simulink model "Local_In"  (R2025b)
settings: Solver=VariableStepAuto  StartTime=0.0  StopTime=10.0  RelTol=1e-3
settings Model: Creator=EMK7KOR  LastModifiedBy=CAQ2KOR

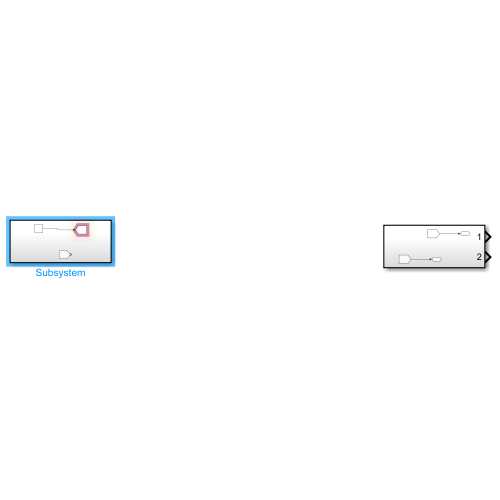
[thumbnail: Simulink's stored preview of the top-level diagram]
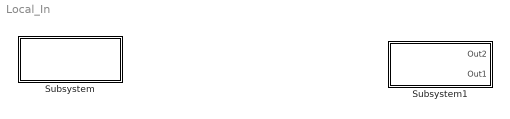
== system Local_In ==
  Subsystem : Subsystem
  Subsystem1 : Subsystem

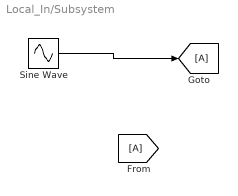
== system Local_In/Subsystem ==
  From : From
  Goto : Goto
  Sine Wave : Sin  SampleTime=0
  wires:
  Sine Wave/1 -> Goto/1

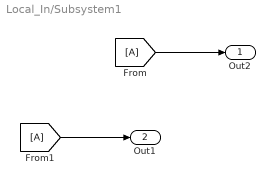
== system Local_In/Subsystem1 ==
  From : From  TagVisibility=global
  From1 : From  TagVisibility=global
  Out2 : Outport
  Out1 : Outport  Port=2
  wires:
  From/1 -> Out2/1
  From1/1 -> Out1/1
